simulink model "fw_mode_manager"  (R2026b)
settings: Solver=VariableStepAuto
undefined symbols (not defined in the file or in its folder): EscState, P, Ts
libraries: simulink x16
settings Model: Creator=aomar  LastModifiedBy=aomar

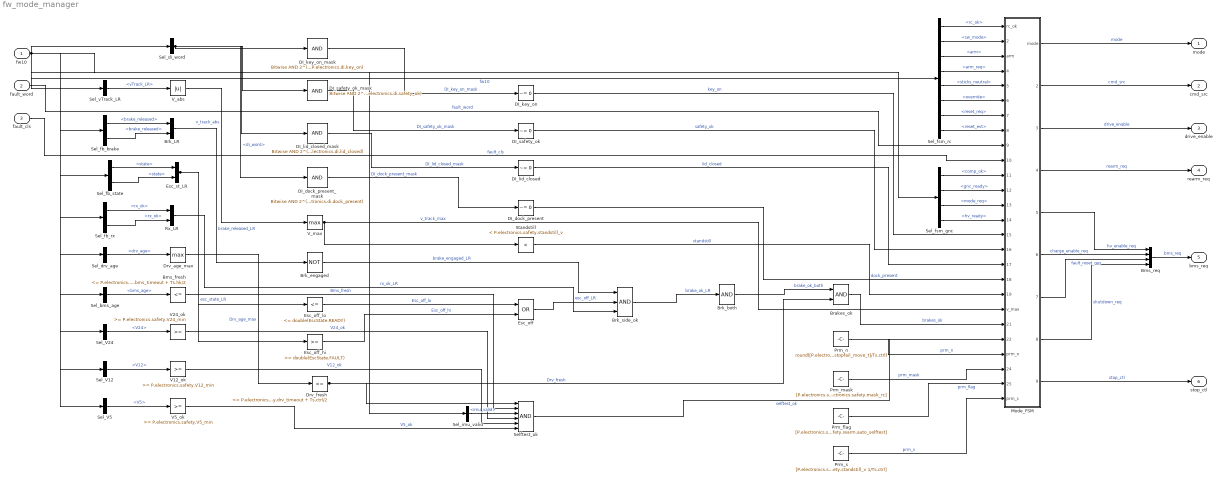
== system fw_mode_manager ==
  fw10 : Inport  SampleTime=Ts.ctrl
  fault_word : Inport  Port=2  OutDataTypeStr=uint32  SampleTime=Ts.ctrl
  fault_cls : Inport  Port=3  OutDataTypeStr=boolean  PortDimensions=3  SampleTime=Ts.ctrl
  Bms_fresh : simulink/Logic and Bit Operations/Compare To Constant  relop=<=  const=P.electronics.safety.bms_timeout + Ts.hk/2  OutDataTypeStr=boolean
  Bms_req : Concatenate  NumInputs=4
  Brakes_ok : Logic  AllPortsSameDT=off  OutDataTypeStr=boolean
  Brk_LR : Concatenate
  Brk_both : Logic  Inputs=1  AllPortsSameDT=off  OutDataTypeStr=boolean
  Brk_engaged : Logic  Operator=NOT  Inputs=1  AllPortsSameDT=off  OutDataTypeStr=boolean
  Brk_side_ok : Logic  Inputs=3  AllPortsSameDT=off  OutDataTypeStr=boolean
  DI_dock_present : simulink/Logic and Bit Operations/Compare To Zero  relop=~=  OutDataTypeStr=boolean
  DI_dock_present_mask : simulink/Logic and Bit Operations/Bitwise Operator  logicop=AND  UseBitMask=on  BitMask=2^(P.electronics.di.dock_present)  BitMaskRealWorld=Stored Integer
  DI_key_on : simulink/Logic and Bit Operations/Compare To Zero  relop=~=  OutDataTypeStr=boolean
  DI_key_on_mask : simulink/Logic and Bit Operations/Bitwise Operator  logicop=AND  UseBitMask=on  BitMask=2^(P.electronics.di.key_on)  BitMaskRealWorld=Stored Integer
  DI_lid_closed : simulink/Logic and Bit Operations/Compare To Zero  relop=~=  OutDataTypeStr=boolean
  DI_lid_closed_mask : simulink/Logic and Bit Operations/Bitwise Operator  logicop=AND  UseBitMask=on  BitMask=2^(P.electronics.di.lid_closed)  BitMaskRealWorld=Stored Integer
  DI_safety_ok : simulink/Logic and Bit Operations/Compare To Zero  relop=~=  OutDataTypeStr=boolean
  DI_safety_ok_mask : simulink/Logic and Bit Operations/Bitwise Operator  logicop=AND  UseBitMask=on  BitMask=2^(P.electronics.di.safety_ok)  BitMaskRealWorld=Stored Integer
  Drv_age_max : MinMax  Function=max
  Drv_fresh : simulink/Logic and Bit Operations/Compare To Constant  relop=<=  const=P.electronics.safety.drv_timeout + Ts.ctrl/2  OutDataTypeStr=boolean
  Esc_off : Logic  Operator=OR  AllPortsSameDT=off  OutDataTypeStr=boolean
  Esc_off_hi : simulink/Logic and Bit Operations/Compare To Constant  relop=>=  const=double(EscState.FAULT)  OutDataTypeStr=boolean
  Esc_off_lo : simulink/Logic and Bit Operations/Compare To Constant  relop=<=  const=double(EscState.READY)  OutDataTypeStr=boolean
  Esc_st_LR : Concatenate
  Mode_FSM : MATLAB Function  TreatAsAtomicUnit=on
  Prm_flag : Constant  Value=[P.electronics.safety.rc_required_in_auto P.electronics.safety.rearm.auto_selftest]  OutDataTypeStr=boolean  SampleTime=Ts.ctrl
  Prm_mask : Constant  Value=[P.electronics.safety.maskA P.electronics.safety.maskB P.electronics.safety.mask_rc]  OutDataTypeStr=uint32  SampleTime=Ts.ctrl
  Prm_n : Constant  Value=round([P.electronics.safety.selftest_t P.electronics.safety.selftest_timeout P.electronics.safety.auto_start_warn_t P.electronics.safety.standstill_t P.electronics.safety.ctrlstop_timeout P.electronics.shaper.estop_tmax P.electronics.safety.stopfail_t0 P.electronics.safety.stopfail_brake_t P.electronics.safety.stopfail_move_t]/Ts.ctrl)  OutDataTypeStr=uint16  SampleTime=Ts.ctrl
  Prm_s : Constant  Value=[P.electronics.shaper.a_ctrlstop P.electronics.shaper.a_estop P.electronics.safety.ctrlstop_t_extra P.electronics.safety.stopfail_dv P.electronics.safety.stopfail_rate P.electronics.safety.standstill_v 1/Ts.ctrl]  OutDataTypeStr=single  SampleTime=Ts.ctrl
  Rx_LR : Concatenate
  Sel_V12 : BusSelector  OutputSignals=adc.V12
  Sel_V24 : BusSelector  OutputSignals=adc.V24
  Sel_V5 : BusSelector  OutputSignals=adc.V5
  Sel_bms_age : BusSelector  OutputSignals=bms_age
  Sel_di_word : BusSelector  OutputSignals=di_word
  Sel_drv_age : BusSelector  OutputSignals=drv_age
  Sel_fb_brake : BusSelector  OutputSignals=drive_fb.L.brake_released,drive_fb.R.brake_released
  Sel_fb_rx : BusSelector  OutputSignals=drive_fb.L.rx_ok,drive_fb.R.rx_ok
  Sel_fb_state : BusSelector  OutputSignals=drive_fb.L.state,drive_fb.R.state
  Sel_fsm_gnc : BusSelector  OutputSignals=comp_ok,gnc_cmd.gnc_ready,gnc_cmd.mode_req,bms.hv_ready
  Sel_fsm_rc : BusSelector  OutputSignals=rc.rc_ok,rc.sw_mode,rc.arm,rc.arm_req,rc.sticks_neutral,rc.override,reset_req,reset_evt
  Sel_imu_valid : BusSelector  OutputSignals=tilt.imu_valid
  Sel_vTrack_LR : BusSelector  OutputSignals=odom.vTrack_LR
  Selftest_ok : Logic  Inputs=6  AllPortsSameDT=off  OutDataTypeStr=boolean
  Standstill : simulink/Logic and Bit Operations/Compare To Constant  relop=<  const=P.electronics.safety.standstill_v  OutDataTypeStr=boolean
  V12_ok : simulink/Logic and Bit Operations/Compare To Constant  relop=>=  const=P.electronics.safety.V12_min  OutDataTypeStr=boolean
  V24_ok : simulink/Logic and Bit Operations/Compare To Constant  relop=>=  const=P.electronics.safety.V24_min  OutDataTypeStr=boolean
  V5_ok : simulink/Logic and Bit Operations/Compare To Constant  relop=>=  const=P.electronics.safety.V5_min  OutDataTypeStr=boolean
  V_abs : Abs  SaturateOnIntegerOverflow=off
  V_max : MinMax  Function=max
  mode : Outport  OutDataTypeStr=uint8
  cmd_src : Outport  Port=2  OutDataTypeStr=uint8
  drive_enable : Outport  Port=3  OutDataTypeStr=boolean
  rearm_req : Outport  Port=4  OutDataTypeStr=boolean
  bms_req : Outport  Port=5  OutDataTypeStr=boolean
  stop_ctl : Outport  Port=6  OutDataTypeStr=boolean
  wires:
  fw10/1 -> Sel_imu_valid/1, Sel_V5/1, Sel_V12/1, Sel_V24/1, Sel_bms_age/1, Sel_drv_age/1, Sel_fb_rx/1, Sel_fsm_gnc/1, Sel_fb_state/1, Sel_fb_brake/1, Sel_vTrack_LR/1, Sel_fsm_rc/1, Sel_di_word/1  "fw10"
  fault_word/1 -> Mode_FSM/9(fault_word)  "fault_word"
  fault_cls/1 -> Mode_FSM/10(fault_cls)  "fault_cls"
  Sel_vTrack_LR/1 -> V_abs/1  "<vTrack_LR>"
  Sel_fb_brake/1 -> Brk_LR/1  "<brake_released>"
  Sel_fb_brake/2 -> Brk_LR/2  "<brake_released>"
  Sel_fb_rx/1 -> Rx_LR/1  "<rx_ok>"
  Sel_fb_rx/2 -> Rx_LR/2  "<rx_ok>"
  Sel_drv_age/1 -> Drv_age_max/1  "<drv_age>"
  Sel_bms_age/1 -> Bms_fresh/1  "<bms_age>"
  Sel_V24/1 -> V24_ok/1  "<V24>"
  Sel_V12/1 -> V12_ok/1  "<V12>"
  Sel_V5/1 -> V5_ok/1  "<V5>"
  Sel_fb_state/1 -> Esc_st_LR/1  "<state>"
  Sel_fb_state/2 -> Esc_st_LR/2  "<state>"
  Sel_di_word/1 -> DI_dock_present_mask/1, DI_lid_closed_mask/1, DI_safety_ok_mask/1, DI_key_on_mask/1  "<di_word>"
  Brk_LR/1 -> Brk_engaged/1  "brake_released_LR"
  Rx_LR/1 -> Brk_side_ok/3  "rx_ok_LR"
  Esc_st_LR/1 -> Esc_off_hi/1, Esc_off_lo/1  "esc_state_LR"
  V_abs/1 -> V_max/1  "v_track_abs"
  Drv_age_max/1 -> Drv_fresh/1  "Drv_age_max"
  Bms_fresh/1 -> Selftest_ok/2  "Bms_fresh"
  V24_ok/1 -> Selftest_ok/4  "V24_ok"
  V12_ok/1 -> Selftest_ok/5  "V12_ok"
  V5_ok/1 -> Selftest_ok/6  "V5_ok"
  V_max/1 -> Mode_FSM/20(v_max), Standstill/1  "v_track_max"
  Brk_engaged/1 -> Brk_side_ok/1  "brake_engaged_LR"
  Esc_off_lo/1 -> Esc_off/1  "Esc_off_lo"
  Esc_off_hi/1 -> Esc_off/2  "Esc_off_hi"
  DI_key_on_mask/1 -> DI_key_on/1  "DI_key_on_mask"
  DI_safety_ok_mask/1 -> DI_safety_ok/1  "DI_safety_ok_mask"
  DI_lid_closed_mask/1 -> DI_lid_closed/1  "DI_lid_closed_mask"
  DI_dock_present_mask/1 -> DI_dock_present/1  "DI_dock_present_mask"
  Drv_fresh/1 -> Brakes_ok/2, Selftest_ok/1  "Drv_fresh"
  Sel_imu_valid/1 -> Selftest_ok/3  "<imu_valid>"
  DI_key_on/1 -> Mode_FSM/15(key_on)  "key_on"
  DI_safety_ok/1 -> Mode_FSM/16(safety_ok)  "safety_ok"
  DI_lid_closed/1 -> Mode_FSM/17(lid_closed)  "lid_closed"
  DI_dock_present/1 -> Mode_FSM/18(dock_present)  "dock_present"
  Standstill/1 -> Mode_FSM/19(standstill)  "standstill"
  Esc_off/1 -> Brk_side_ok/2  "esc_off_LR"
  Selftest_ok/1 -> Mode_FSM/22(selftest_ok)  "selftest_ok"
  Brk_side_ok/1 -> Brk_both/1  "brake_ok_LR"
  Brk_both/1 -> Brakes_ok/1  "brake_ok_both"
  Brakes_ok/1 -> Mode_FSM/21(brakes_ok)  "brakes_ok"
  Prm_n/1 -> Mode_FSM/23(prm_n)  "prm_n"
  Prm_mask/1 -> Mode_FSM/24(prm_mask)  "prm_mask"
  Prm_flag/1 -> Mode_FSM/25(prm_flag)  "prm_flag"
  Prm_s/1 -> Mode_FSM/26(prm_s)  "prm_s"
  Sel_fsm_rc/1 -> Mode_FSM/1(rc_ok)  "<rc_ok>"
  Sel_fsm_rc/2 -> Mode_FSM/2(sw_mode)  "<sw_mode>"
  Sel_fsm_rc/3 -> Mode_FSM/3(arm)  "<arm>"
  Sel_fsm_rc/4 -> Mode_FSM/4(arm_req)  "<arm_req>"
  Sel_fsm_rc/5 -> Mode_FSM/5(sticks_neutral)  "<sticks_neutral>"
  Sel_fsm_rc/6 -> Mode_FSM/6(override)  "<override>"
  Sel_fsm_rc/7 -> Mode_FSM/7(reset_req)  "<reset_req>"
  Sel_fsm_rc/8 -> Mode_FSM/8(reset_evt)  "<reset_evt>"
  Sel_fsm_gnc/1 -> Mode_FSM/11(comp_ok)  "<comp_ok>"
  Sel_fsm_gnc/2 -> Mode_FSM/12(gnc_ready)  "<gnc_ready>"
  Sel_fsm_gnc/3 -> Mode_FSM/13(mode_req)  "<mode_req>"
  Sel_fsm_gnc/4 -> Mode_FSM/14(hv_ready)  "<hv_ready>"
  Mode_FSM/1(mode) -> mode/1  "mode"
  Mode_FSM/2(cmd_src) -> cmd_src/1  "cmd_src"
  Mode_FSM/3(drive_enable) -> drive_enable/1  "drive_enable"
  Mode_FSM/4(rearm_req) -> rearm_req/1  "rearm_req"
  Mode_FSM/5(hv_req) -> Bms_req/1  "hv_enable_req"
  Mode_FSM/6(chg_req) -> Bms_req/2  "charge_enable_req"
  Mode_FSM/7(rst_req) -> Bms_req/3  "fault_reset_req"
  Mode_FSM/8(off_req) -> Bms_req/4  "shutdown_req"
  Mode_FSM/9(stop_ctl) -> stop_ctl/1  "stop_ctl"
  Bms_req/1 -> bms_req/1  "bms_req"

== matlab function fw_mode_manager/Mode_FSM ==
  settings: description=MCU mode manager FSM (T09). Constants arrive on inputs (no parameter data).
  data: rc_ok input; mode output; sw_mode input; arm input; arm_req input; sticks_neutral input; override input; reset_req input; reset_evt input; fault_word input; fault_cls input; comp_ok input; gnc_ready input; mode_req input; hv_ready input; key_on input; safety_ok input; lid_closed input; dock_present input; standstill input; v_max input; brakes_ok input; selftest_ok input; prm_n input; prm_mask input; prm_flag input; prm_s input; cmd_src output; drive_enable output; rearm_req output; hv_req output; chg_req output; rst_req output; off_req output; stop_ctl output
function [mode, cmd_src, drive_enable, rearm_req, hv_req, chg_req, rst_req, off_req, stop_ctl] = fcn(rc_ok, sw_mode, arm, arm_req, sticks_neutral, override, reset_req, reset_evt, fault_word, fault_cls, comp_ok, gnc_ready, mode_req, hv_ready, key_on, safety_ok, lid_closed, dock_present, standstill, v_max, brakes_ok, selftest_ok, prm_n, prm_mask, prm_flag, prm_s)
%#codegen
% body: subsystems/electronics/mcu_mode_manager.m (ShaddadMode FSM, T09); bms_req leaves as 4 scalars
[mode, cmd_src, drive_enable, rearm_req, bms_req, stop_ctl] = mcu_mode_manager(rc_ok, sw_mode, arm, arm_req, sticks_neutral, override, reset_req, reset_evt, fault_word, fault_cls, comp_ok, gnc_ready, mode_req, hv_ready, key_on, safety_ok, lid_closed, dock_present, standstill, v_max, brakes_ok, selftest_ok, prm_n, prm_mask, prm_flag, prm_s);
hv_req = bms_req(1); chg_req = bms_req(2); rst_req = bms_req(3); off_req = bms_req(4);
